simulink model "observador_de_estado_reducido_retroalimentacion_integral"  (R2026b)
settings: Solver=VariableStepAuto
values from neighbouring files (symbols this model uses):
  J_eq = J_m + J_l/(r^2)    (= 2.84652777778e-05)    [coeficientes.m]
  K_ei = p_obs^3    (= 32768000000)    [coeficientes.m]
  K_et = 2*p_obs    (= 6400)    [coeficientes.m]
  K_ew = p_obs^2    (= 10240000)    [coeficientes.m]
settings Model: Creator=lamun  LastModifiedBy=lamun

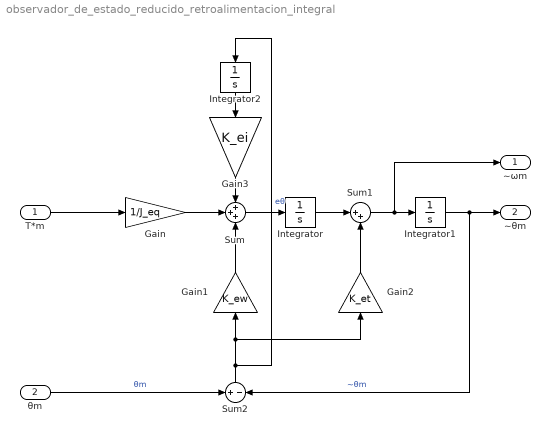
== system observador_de_estado_reducido_retroalimentacion_integral ==
  T*m : Inport
  θm : Inport  Port=2
  Gain : Gain  Gain=1/J_eq
  Gain1 : Gain  Gain=K_ew
  Gain2 : Gain  Gain=K_et
  Gain3 : Gain  Gain=K_ei
  Integrator : Integrator
  Integrator1 : Integrator
  Integrator2 : Integrator
  Sum : Sum  Inputs=+++
  Sum1 : Sum  Inputs=|++
  Sum2 : Sum  Inputs=+-
  ~ωm : Outport
  ~θm : Outport  Port=2
  wires:
  Sum2/1 -> Integrator2/1, Gain2/1, Gain1/1  "eθ"
  T*m/1 -> Gain/1
  Gain2/1 -> Sum1/2
  Gain/1 -> Sum/2
  Gain1/1 -> Sum/3
  Sum1/1 -> ~ωm/1, Integrator1/1
  Sum/1 -> Integrator/1
  Integrator/1 -> Sum1/1
  θm/1 -> Sum2/1  "θm"
  Integrator1/1 -> Sum2/2, ~θm/1  "~θm"
  Integrator2/1 -> Gain3/1
  Gain3/1 -> Sum/1
